simulink model "Es2_stateflow"  (R2025b)
settings: Solver=VariableStepAuto  StartTime=0.0  StopTime=7  RelTol=1e-3
settings Model: Creator=fsisa  LastModifiedBy=fsisa

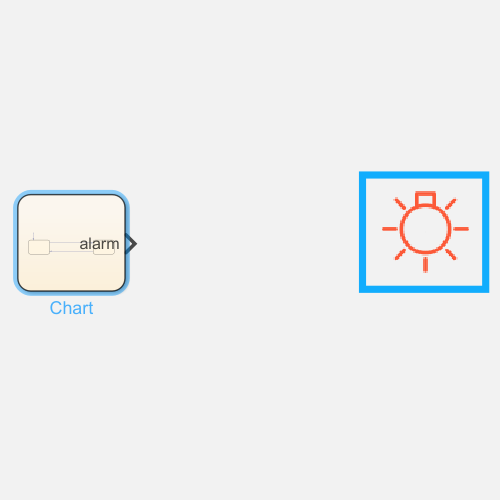
[thumbnail: Simulink's stored preview of the top-level diagram]
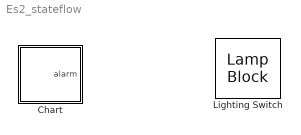
== system Es2_stateflow ==
  Chart : Stateflow chart  TreatAsAtomicUnit=on
  Lighting Switch : LampBlock  LabelPosition=Hide  DefaultColor=[192.0, 192.0, 192.0]  Icon=LightingSwitch

== stateflow chart Es2_stateflow/Chart ==
  state DISACTIVATE
    entry:
    alarm=0
  state ACTIVATE
    entry:
    alarm=1
  (default) -> DISACTIVATE
  DISACTIVATE -> ACTIVATE : after(1,sec)
  ACTIVATE -> DISACTIVATE : after(5, sec)
  data: alarm output
